simulink model "schuler_loop"  (Simulink 7.5)
settings: Solver=ode45  StartTime=0.0  StopTime=5040  RelTol=1e-3
libraries: simulink x4
settings Model: Creator=carrollmic  LastModifiedBy=carrollmic
settings OptimizationCC: BlockReduction=off  BooleanDataType=off
settings DebuggingCC: SaveWithParameterizedLinksMsg=none  SignalResolutionControl=TryResolveAllWithWarning  SolverPrmCheckMsg=none  MultiTaskDSMMsg=warning  MultiTaskCondExecSysMsg=none  StrictBusMsg=None
settings HardwareCC: TargetUnknown=on
settings RTWCC: IncludeERTFirstTime=on

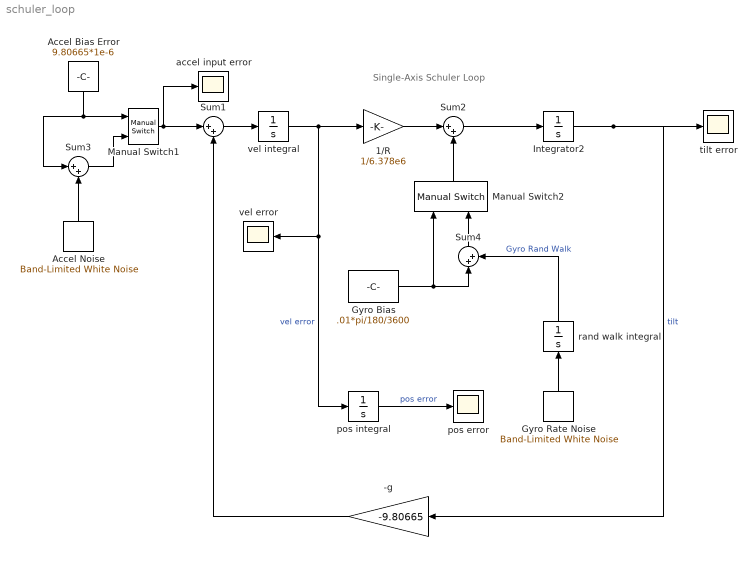
== system schuler_loop ==
  note: Single-Axis Schuler Loop
  -g : Gain  Gain=-9.80665  SaturateOnIntegerOverflow=on  OutDataTypeStr=Inherit: Same as input  ParamDataTypeStr=Inherit: Same as input
  1/R : Gain  Gain=1/6.378e6  SaturateOnIntegerOverflow=on  OutDataTypeStr=Inherit: Same as input  ParamDataTypeStr=Inherit: Same as input
  Accel Bias Error : Constant  Value=9.80665*1e-6
  Accel Noise : simulink/Sources/Band-Limited White Noise  SystemSampleTime=-1  Cov=[9.80665*1e-6]  Ts=0.1  seed=[23341]
  Gyro Bias : Constant  Value=.01*pi/180/3600
  Gyro Rate Noise : simulink/Sources/Band-Limited White Noise  SystemSampleTime=-1  Cov=[0.0001^2*(pi/180)/3600]  Ts=0.1  seed=[23341]
  Integrator2 : Integrator
  Manual Switch1 : simulink/Signal Routing/Manual Switch  SystemSampleTime=-1  sw=0  action=0  varsize=off
  Manual Switch2 : simulink/Signal Routing/Manual Switch  SystemSampleTime=-1  sw=1  action=0  varsize=off
  Sum{1..4} (4 alike) : Sum  Inputs=|++  SaturateOnIntegerOverflow=on  InputSameDT=on  OutDataTypeStr=Inherit: Same as first input
  accel input error : Scope
      settings: YMin=-30000  YMax=2500  SaveName=ScopeData3  MaxDataPoints=5040
  pos error : Scope
      settings: TimeRange=5040  YMin=-2000  YMax=250  MaxDataPoints=5040  SampleInput=on  SampleTime=1
  pos integral : Integrator
  rand walk integral : Integrator
  "tilt error " : Scope
      settings: TimeRange=5040  YMin=-0.25  YMax=4  MaxDataPoints=5400  SampleInput=on  SampleTime=1
  vel error : Scope
      settings: YMin=-30000  YMax=2500  SaveName=ScopeData2  MaxDataPoints=5040
  vel integral : Integrator
  wires:
  Sum2/1 -> Integrator2/1
  -g/1 -> Sum1/2
  Sum1/1 -> vel integral/1
  vel integral/1 -> 1/R/1, pos integral/1, vel error/1  "vel error"
  1/R/1 -> Sum2/1
  Manual Switch1/1 -> Sum1/1, accel input error/1
  Accel Noise/1 -> Sum3/2
  Accel Bias Error/1 -> Sum3/1, Manual Switch1/1
  Sum3/1 -> Manual Switch1/2
  Integrator2/1 -> "tilt error "/1, -g/1  "tilt"
  Gyro Bias/1 -> Manual Switch2/1, Sum4/1
  rand walk integral/1 -> Sum4/2  "Gyro Rand Walk"
  Gyro Rate Noise/1 -> rand walk integral/1
  Sum4/1 -> Manual Switch2/2
  pos integral/1 -> pos error/1  "pos error"
  Manual Switch2/1 -> Sum2/2
